simulink subsystem "Odometry_sub"  (R2023b)
settings: Solver=VariableStepAuto  StartTime=0.0  StopTime=10.0  RelTol=1e-3
undefined symbols (not defined in the file): Odometry_IC_X, Odometry_IC_Y
settings Model: Creator=ander  LastModifiedBy=ander

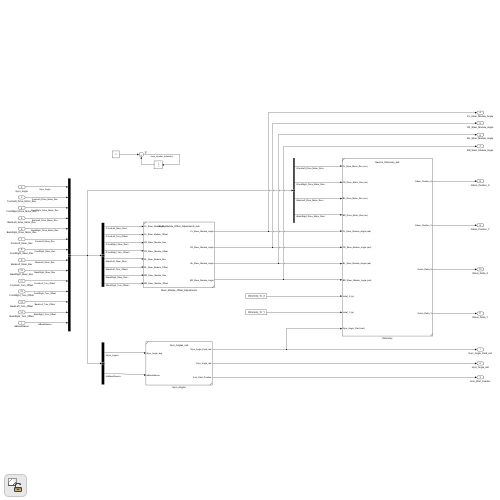
[thumbnail: Simulink's stored preview of the top-level diagram]
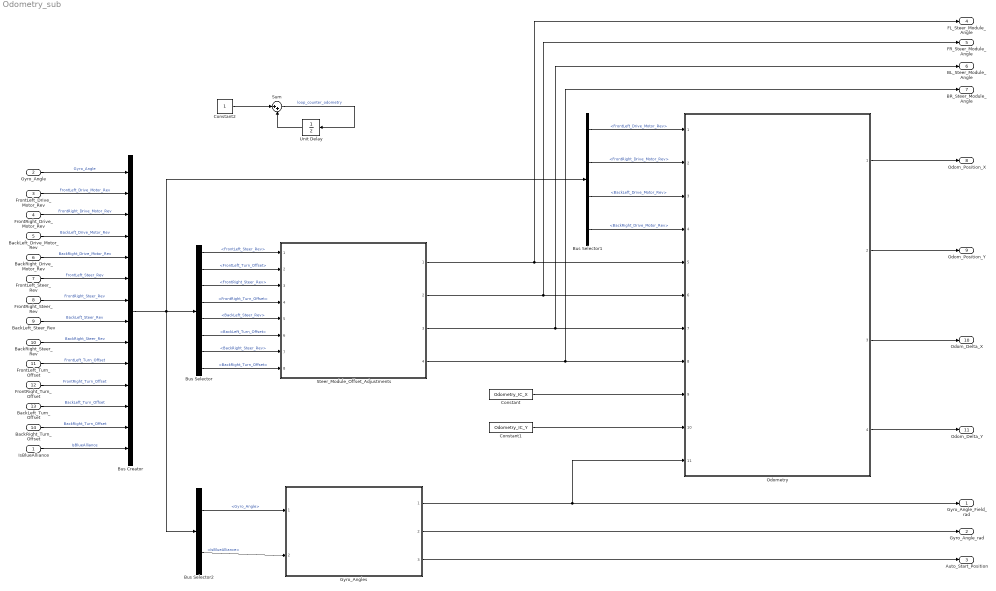
== system Odometry_sub ==
  IsBlueAlliance : Inport
  Gyro_Angle : Inport  Port=2
  FrontLeft_Drive_Motor_Rev : Inport  Port=3
  FrontRight_Drive_Motor_Rev : Inport  Port=4
  BackLeft_Drive_Motor_Rev : Inport  Port=5
  BackRight_Drive_Motor_Rev : Inport  Port=6
  FrontLeft_Steer_Rev : Inport  Port=7
  FrontRight_Steer_Rev : Inport  Port=8
  BackLeft_Steer_Rev : Inport  Port=9
  BackRight_Steer_Rev : Inport  Port=10
  FrontLeft_Turn_Offset : Inport  Port=11
  FrontRight_Turn_Offset : Inport  Port=12
  BackLeft_Turn_Offset : Inport  Port=13
  BackRight_Turn_Offset : Inport  Port=14
  Bus Creator : BusCreator  Inputs=14
  Bus Selector : BusSelector  OutputSignals=FrontLeft_Steer_Rev,FrontLeft_Turn_Offset,FrontRight_Steer_Rev,FrontRight_Turn_Offset,BackLeft_Steer_Rev,BackLeft_Turn_Offset,BackRight_Steer_Rev,BackRight_Turn_Offset
  Bus Selector1 : BusSelector  OutputSignals=FrontLeft_Drive_Motor_Rev,FrontRight_Drive_Motor_Rev,BackLeft_Drive_Motor_Rev,BackRight_Drive_Motor_Rev
  Bus Selector2 : BusSelector  OutputSignals=Gyro_Angle,IsBlueAlliance
  Constant : Constant  Value=Odometry_IC_X
  Constant1 : Constant  Value=Odometry_IC_Y
  Constant2 : Constant
  Gyro_Angles : Subsystem  ReferencedSubsystem=Gyro_Angles_sub
  Odometry : Subsystem  ReferencedSubsystem=Swerve_Odometry_sub
  Steer_Module_Offset_Adjustments : Subsystem  ReferencedSubsystem=Steer_Module_Offset_Adjustments_sub
  Sum : Sum  Inputs=|++
  Unit Delay : UnitDelay  SampleTime=-1  HasFrameUpgradeWarning=on
  Gyro_Angle_Field_rad : Outport
  Gyro_Angle_rad : Outport  Port=2
  Auto_Start_Position : Outport  Port=3
  FL_Steer_Module_Angle : Outport  Port=4  OutDataTypeStr=double  Unit=rad
  FR_Steer_Module_Angle : Outport  Port=5  OutDataTypeStr=double  Unit=rad
  BL_Steer_Module_Angle : Outport  Port=6  OutDataTypeStr=double  Unit=rad
  BR_Steer_Module_Angle : Outport  Port=7  OutDataTypeStr=double  Unit=rad
  Odom_Position_X : Outport  Port=8
  Odom_Position_Y : Outport  Port=9
  Odom_Delta_X : Outport  Port=10
  Odom_Delta_Y : Outport  Port=11
  wires:
  Constant/1 -> Odometry/9
  Constant1/1 -> Odometry/10
  Gyro_Angles/1 -> Gyro_Angle_Field_rad/1, Odometry/11
  Steer_Module_Offset_Adjustments/1 -> Odometry/5, FL_Steer_Module_Angle/1
  Steer_Module_Offset_Adjustments/2 -> Odometry/6, FR_Steer_Module_Angle/1
  Steer_Module_Offset_Adjustments/3 -> Odometry/7, BL_Steer_Module_Angle/1
  Steer_Module_Offset_Adjustments/4 -> Odometry/8, BR_Steer_Module_Angle/1
  Odometry/1 -> Odom_Position_X/1
  Odometry/2 -> Odom_Position_Y/1
  Odometry/3 -> Odom_Delta_X/1
  Odometry/4 -> Odom_Delta_Y/1
  Gyro_Angles/2 -> Gyro_Angle_rad/1
  BackRight_Turn_Offset/1 -> Bus Creator/13  "BackRight_Turn_Offset"
  BackLeft_Turn_Offset/1 -> Bus Creator/12  "BackLeft_Turn_Offset"
  FrontRight_Turn_Offset/1 -> Bus Creator/11  "FrontRight_Turn_Offset"
  FrontLeft_Turn_Offset/1 -> Bus Creator/10  "FrontLeft_Turn_Offset"
  BackRight_Steer_Rev/1 -> Bus Creator/9  "BackRight_Steer_Rev"
  BackLeft_Steer_Rev/1 -> Bus Creator/8  "BackLeft_Steer_Rev"
  FrontRight_Steer_Rev/1 -> Bus Creator/7  "FrontRight_Steer_Rev"
  FrontLeft_Steer_Rev/1 -> Bus Creator/6  "FrontLeft_Steer_Rev"
  BackRight_Drive_Motor_Rev/1 -> Bus Creator/5  "BackRight_Drive_Motor_Rev"
  BackLeft_Drive_Motor_Rev/1 -> Bus Creator/4  "BackLeft_Drive_Motor_Rev"
  FrontRight_Drive_Motor_Rev/1 -> Bus Creator/3  "FrontRight_Drive_Motor_Rev"
  FrontLeft_Drive_Motor_Rev/1 -> Bus Creator/2  "FrontLeft_Drive_Motor_Rev"
  Gyro_Angle/1 -> Bus Creator/1  "Gyro_Angle"
  Bus Creator/1 -> Bus Selector/1, Bus Selector2/1, Bus Selector1/1
  Bus Selector/5 -> Steer_Module_Offset_Adjustments/5  "<BackLeft_Steer_Rev>"
  Bus Selector/4 -> Steer_Module_Offset_Adjustments/4  "<FrontRight_Turn_Offset>"
  Bus Selector/6 -> Steer_Module_Offset_Adjustments/6  "<BackLeft_Turn_Offset>"
  Bus Selector/3 -> Steer_Module_Offset_Adjustments/3  "<FrontRight_Steer_Rev>"
  Bus Selector/7 -> Steer_Module_Offset_Adjustments/7  "<BackRight_Steer_Rev>"
  Bus Selector/2 -> Steer_Module_Offset_Adjustments/2  "<FrontLeft_Turn_Offset>"
  Bus Selector/8 -> Steer_Module_Offset_Adjustments/8  "<BackRight_Turn_Offset>"
  Bus Selector/1 -> Steer_Module_Offset_Adjustments/1  "<FrontLeft_Steer_Rev>"
  Bus Selector1/1 -> Odometry/1  "<FrontLeft_Drive_Motor_Rev>"
  Bus Selector1/2 -> Odometry/2  "<FrontRight_Drive_Motor_Rev>"
  Bus Selector1/3 -> Odometry/3  "<BackLeft_Drive_Motor_Rev>"
  Bus Selector1/4 -> Odometry/4  "<BackRight_Drive_Motor_Rev>"
  Bus Selector2/1 -> Gyro_Angles/1  "<Gyro_Angle>"
  IsBlueAlliance/1 -> Bus Creator/14  "IsBlueAlliance"
  Bus Selector2/2 -> Gyro_Angles/2  "<IsBlueAlliance>"
  Gyro_Angles/3 -> Auto_Start_Position/1
  Constant2/1 -> Sum/1
  Sum/1 -> Unit Delay/1  "loop_counter_odometry"
  Unit Delay/1 -> Sum/2
